simulink model "fi_cc"  (R2026a)
settings: Solver=VariableStepAuto  StartTime=0  StopTime=100  FixedStep=0.1  MinStep=0.01  AbsTol=1e-5  EnableMultiTasking=on
settings Model: Creator=yoriyuki  LastModifiedBy=harry_31916
settings DataIOCC: ExternalInput=[Throttle, Brake]  FinalStateName=SavePoint  InitialState=SavePoint  SaveOperatingPoint=on  StateSaveName=x  TimeSaveName=t  OutputSaveName=y

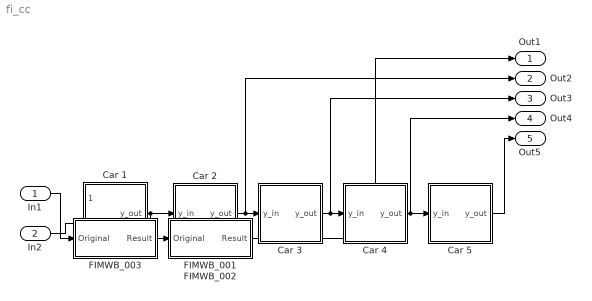
== system fi_cc ==
  In1 : Inport
  In2 : Inport  Port=2
  Car 1 : Stateflow chart  TreatAsAtomicUnit=on
  Car 2 : Stateflow chart  TreatAsAtomicUnit=on
  Car 3 : Stateflow chart  TreatAsAtomicUnit=on
  Car 4 : Stateflow chart  TreatAsAtomicUnit=on
  Car 5 : Stateflow chart  TreatAsAtomicUnit=on
  FIMWB_001 : Subsystem  Tag=fimwb.fault.1
  FIMWB_002 : Subsystem  Tag=fimwb.fault.2
  FIMWB_003 : Subsystem  Tag=fimwb.fault.3
  Out1 : Outport  VectorParamsAs1DForOutWhenUnconnected=off
  Out2 : Outport  Port=2  VectorParamsAs1DForOutWhenUnconnected=off
  Out3 : Outport  Port=3  VectorParamsAs1DForOutWhenUnconnected=off
  Out4 : Outport  Port=4  VectorParamsAs1DForOutWhenUnconnected=off
  Out5 : Outport  Port=5  VectorParamsAs1DForOutWhenUnconnected=off
  wires:
  Car 5/1(y_out) -> Out5/1
  Car 1/1(y_out) -> Car 2/1(y_in), FIMWB_001/1(Original)
  Car 2/1(y_out) -> Out2/1, Car 3/1(y_in)
  Car 3/1(y_out) -> Out3/1, Car 4/1(y_in)
  Car 4/1(y_out) -> Car 5/1(y_in), Out4/1
  In2/1 -> Car 1/2(Brake)
  FIMWB_001/1(Result) -> FIMWB_002/1(Original)
  FIMWB_002/1(Result) -> Out1/1
  In1/1 -> FIMWB_003/1(Original)
  FIMWB_003/1(Result) -> Car 1/1(Throttle)

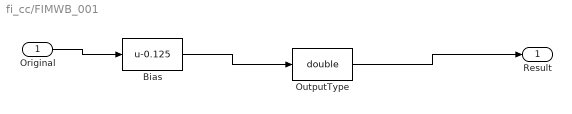
== system fi_cc/FIMWB_001 ==
  Original : Inport
  Bias : Bias  Bias=-0.125  SaturateOnIntegerOverflow=off
  OutputType : DataTypeConversion  OutDataTypeStr=double  RndMeth=Round
  Result : Outport
  wires:
  Original/1 -> Bias/1
  Bias/1 -> OutputType/1
  OutputType/1 -> Result/1

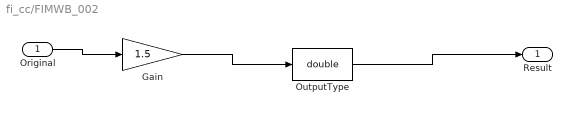
== system fi_cc/FIMWB_002 ==
  Original : Inport
  Gain : Gain  Gain=1.5  OutDataTypeStr=Inherit: Same as input
  OutputType : DataTypeConversion  OutDataTypeStr=double  RndMeth=Round
  Result : Outport
  wires:
  Original/1 -> Gain/1
  Gain/1 -> OutputType/1
  OutputType/1 -> Result/1

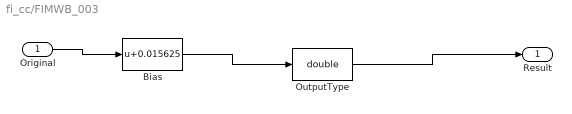
== system fi_cc/FIMWB_003 ==
  Original : Inport
  Bias : Bias  Bias=0.015625  SaturateOnIntegerOverflow=off
  OutputType : DataTypeConversion  OutDataTypeStr=double  RndMeth=Round
  Result : Outport
  wires:
  Original/1 -> Bias/1
  Bias/1 -> OutputType/1
  OutputType/1 -> Result/1

== stateflow chart fi_cc/Car 1 ==
  settings: updateMethod=CONTINUOUS
  state Run
    during:
    v_dot = -Throttle - Brake * v;
    y_dot = v;
    y_out = y;
  (default) -> Run
  data: Throttle input; Brake input; y local =0; y_out output; v local =0
  data y settings: updateMethod=SF_CONTINUOUS_TIME_DATA
  data v settings: updateMethod=SF_CONTINUOUS_TIME_DATA

== stateflow chart fi_cc/Car 3 ==
  settings: updateMethod=CONTINUOUS
  state Chasing
    during:
    v_dot = 1;
    y_dot = -v;
    y_out = y;
  state Keeping
    during:
    y_dot = v;
    y_out = y;
  state Braking
    during:
    v_dot = -v;
    y_dot = -v;
    y_out = y;
  (default) -> Keeping
  Chasing -> Keeping : [y - y_in <= 10]
      | % [transition condition]{action}
  Keeping -> Chasing [order 1] : [y - y_in >=15]
  Braking -> Chasing : [y - y_in >= 20]
  Keeping -> Braking [order 2] : [y - y_in <=5]
  data: y_out output; y local double =20; v local =0; y_in input
  data y settings: updateMethod=SF_CONTINUOUS_TIME_DATA
  data v settings: updateMethod=SF_CONTINUOUS_TIME_DATA
  data y_in settings: updateMethod=SF_CONTINUOUS_TIME_DATA

== stateflow chart fi_cc/Car 2 ==
  settings: updateMethod=CONTINUOUS
  state Chasing
    during:
    v_dot = 1;
    y_dot = -v;
    y_out = y;
  state Keeping
    during:
    y_dot = v;
    y_out = y;
  state Braking
    during:
    v_dot = -v;
    y_dot = -v;
    y_out = y;
  (default) -> Keeping
  Chasing -> Keeping : [y - y_in <= 10]
  Keeping -> Chasing [order 1] : [y - y_in >=15]
  Braking -> Chasing : [y - y_in >= 20]
  Keeping -> Braking [order 2] : [y - y_in <=5]
  data: y_out output; y local double =10; v local =0; y_in input
  data y settings: updateMethod=SF_CONTINUOUS_TIME_DATA
  data v settings: updateMethod=SF_CONTINUOUS_TIME_DATA
  data y_in settings: updateMethod=SF_CONTINUOUS_TIME_DATA

== stateflow chart fi_cc/Car 4 ==
  settings: updateMethod=CONTINUOUS
  state Chasing
    during:
    v_dot = 1;
    y_dot = -v;
    y_out = y;
  state Keeping
    during:
    y_dot = v;
    y_out = y;
  state Braking
    during:
    v_dot = -v;
    y_dot = -v;
    y_out = y;
  (default) -> Keeping
  Chasing -> Keeping : [y - y_in <= 10]
      | % [transition condition]{action}
  Keeping -> Chasing [order 1] : [y - y_in >=15]
  Braking -> Chasing : [y - y_in >= 20]
  Keeping -> Braking [order 2] : [y - y_in <=5]
  data: y local double =30; v local =0; y_in input; y_out output
  data y settings: updateMethod=SF_CONTINUOUS_TIME_DATA
  data v settings: updateMethod=SF_CONTINUOUS_TIME_DATA
  data y_in settings: updateMethod=SF_CONTINUOUS_TIME_DATA

== stateflow chart fi_cc/Car 5 ==
  settings: updateMethod=CONTINUOUS
  state Keeping
    during:
    y_dot = v;
    y_out = y;
  state Chasing
    during:
    v_dot = 1;
    y_dot = -v;
    y_out = y;
  state Braking
    during:
    v_dot = -v;
    y_dot = -v;
    y_out = y;
  (default) -> Keeping
  Chasing -> Keeping : [y - y_in <= 10]
      | % [transition condition]{action}
  Keeping -> Chasing [order 1] : [y - y_in >=15]
  Braking -> Chasing : [y - y_in >= 20]
  Keeping -> Braking [order 2] : [y - y_in <=5]
  data: y_out output; y local double =40; v local =0; y_in input
  data y settings: updateMethod=SF_CONTINUOUS_TIME_DATA
  data v settings: updateMethod=SF_CONTINUOUS_TIME_DATA
  data y_in settings: updateMethod=SF_CONTINUOUS_TIME_DATA
